simulink model "faultdetection"  (R2024b)
settings: Solver=VariableStepAuto  StartTime=0.0  StopTime=0.7  RelTol=1e-3
libraries: spsThreePhaseFaultLib x6, spsThreePhaseSourceLib x3, spsDistributedParametersLineLib x2, spsGroundLib x2, spsThreePhaseParallelRLCLoadLib x2, spsThreePhaseTransformer12TerminalsLib x2, spsThreePhaseSeriesRLCLoadLib x1, spsThreePhaseVIMeasurementLib x1, spspowerguiLib x1
settings Model: Creator=Vignesh  LastModifiedBy=Vignesh

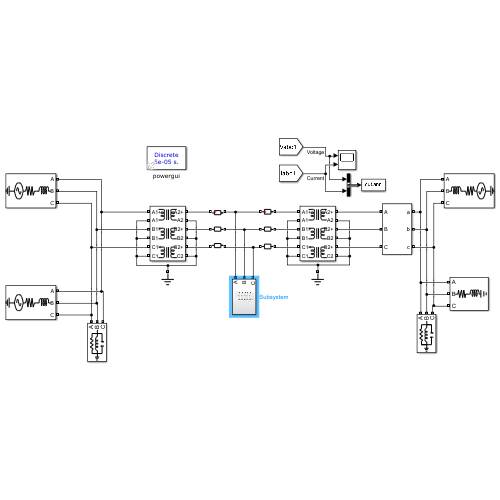
[thumbnail: Simulink's stored preview of the top-level diagram]
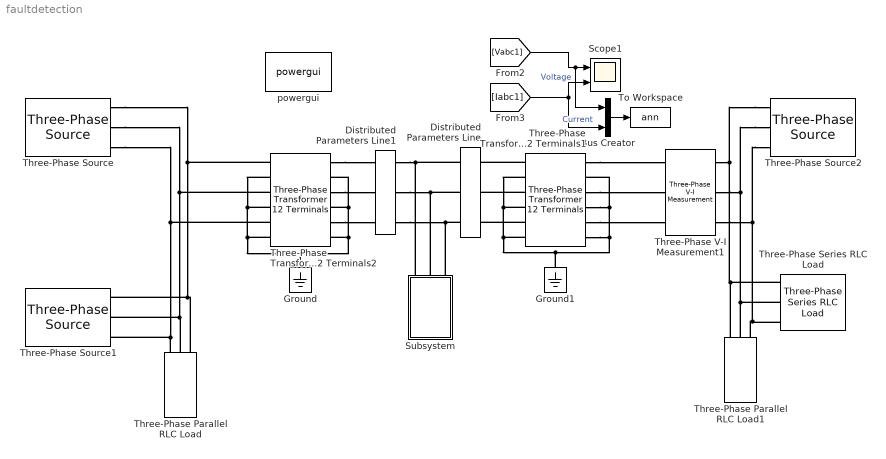
== system faultdetection ==
  Bus Creator : BusCreator  Inputs=2
  Distributed Parameters Line : spsDistributedParametersLineLib/Distributed Parameters Line  Phases=3  Length=33  Frequency=50  Resistance=[0.0132 0.132]  Inductance="[0.9337e-3  4.1264e-3]"  Capacitance=[12.74e-9 7.751e-9]  x1=[-0.0002 1.41144342231724e-10 0 0;-0.00015 1.41380923094757e-10 15635.7791244008 -78733.8101924467;-0.0001 1.41582620330545e-10 16870.5471169943 -78478.5008535494;-5e-05 1.41749384173313e-10 18101.1525545262 -78203.8281188655]  x2=[-0.0002 1.6678837341959e-10 0 0;-0.00015 1.66989876734227e-10 15586.3909292956 -78738.6897884685;-0.0001 1.67150177795504e-10 16821.2416601512 -78484.1556036395;-5e-05 1.67269237051531e-10 18051.9420013289 -78210.256627799]  x3=[-0.0002 9.38203448664615e-13 0 0;-0.00015 9.44868320985513e-13 51.7591743809092 -286.446961708197;-0.0001 9.51300061186575e-13 56.2521023005721 -285.598625681596;-5e-05 9.57497082332148e-13 60.7311508557105 -284.679822467613]  x4=[-0.0002 4.33487932405732e-13 0 0;-0.00015 4.17361641657976e-13 53.0400736803456 -296.594100248532;-0.0001 4.01132373170257e-13 57.6922279035007 -295.724392902891;-5e-05 3.84804131271731e-13 62.330147432688 -294.78171998832]  x5=0.000186628717108595  V1=[2.547e-09 1.32e+05 1.32e+05;314.2 314.2 314.2;-0.1043 0.8095 -0.7613]  V2=[2.522e-09 1.32e+05 1.32e+05;314.2 314.2 314.2;-0.1193 0.8007 -0.7701]  I1=[2.615e-12 367.2 367.2;314.2 314.2 314.2;-0.5343 0.7771 -0.7937]  I2=[5.144e-12 607 607;314.2 314.2 314.2;-0.488 0.7934 -0.7774]  nHarmo=1  Measurements=None  Decoupling=off  VsMag0=0  VrMag0=0  VsAngle0=0  VrAngle0=0  IsMag0=0  IrMag0=0  IsAngle0=0  IrAngle0=0
      settings: LibrarySourceBlock=sps_lib/Power Grid Elements/Distributed Parameters Line
  Distributed Parameters Line1 : spsDistributedParametersLineLib/Distributed Parameters Line  Phases=3  Length=33  Frequency=50  Resistance=[0.0132 0.132]  Inductance="[0.9337e-3  4.1264e-3]"  Capacitance=[12.74e-9 7.751e-9]  x1=[-0.0002 1.51351450754522e-10 0 0;-0.00015 1.51768626873871e-10 15674.3204924212 -78626.6776409923;-0.0001 1.52148356355501e-10 16907.4009652817 -78370.7761372749;-5e-05 1.52490545506846e-10 18136.3097899449 -78095.5378172326]  x2=[-0.0002 1.41144342231724e-10 0 0;-0.00015 1.41380923094757e-10 15635.7791244008 -78733.8101924467;-0.0001 1.41582620330545e-10 16870.5471169943 -78478.5008535494;-5e-05 1.41749384173313e-10 18101.1525545262 -78203.8281188655]  x3=[-0.0002 9.38648272335829e-13 0 0;-0.00015 9.45202034808867e-13 41.4228708035807 -287.645866206956;-0.0001 9.51522582823177e-13 45.9359054607534 -286.959737874603;-5e-05 9.57608356878114e-13 50.4376061206073 -286.202806520801]  x4=[-0.0002 -6.45314572399451e-13 0 0;-0.00015 -6.40074957863135e-13 63.708177517745 -294.987739785218;-0.0001 -6.34677414408614e-13 68.3337840298898 -293.950663320191;-5e-05 -6.2912327379897e-13 72.9425302033256 -292.841058927468]  x5=0.000186628717108595  V1=[2.618e-09 1.319e+05 1.319e+05;314.2 314.2 314.2;-0.1003 0.8184 -0.7524]  V2=[2.549e-09 1.32e+05 1.32e+05;314.2 314.2 314.2;-0.1043 0.8095 -0.7613]  I1=[2.387e-12 367.3 367.3;314.2 314.2 314.2;0.1434 0.7414 -0.8294]  I2=[6.175e-12 607.4 607.4;314.2 314.2 314.2;-0.4569 0.8292 -0.7416]  nHarmo=1  Measurements=None  Decoupling=off  VsMag0=0  VrMag0=0  VsAngle0=0  VrAngle0=0  IsMag0=0  IrMag0=0  IsAngle0=0  IrAngle0=0
      settings: LibrarySourceBlock=sps_lib/Power Grid Elements/Distributed Parameters Line
  Ground : spsGroundLib/Ground  LConnTagsString=a
  Ground1 : spsGroundLib/Ground  LConnTagsString=a
  Scope1 : Scope  NumInputPorts=2
  Subsystem : Subsystem
  Three-Phase Parallel RLC Load : spsThreePhaseParallelRLCLoadLib/Three-Phase Parallel RLC Load  LConnTagsString=A|B|C  Configuration=Y (grounded)  NominalVoltage=1000  Vabc=[1e3 1e3 1e3]  Vabcp=[1e3 1e3 1e3]  NominalFrequency=60  UnbalancedPower=off  ActivePower=10e4  InductivePower=100  CapacitivePower=100  Pabc=[10e3 9e3 11e3]  QLabc=[100 90 110]  QCabc=[100 90 110]  Pabcp=[10e3 9e3 11e3]  QLabcp=[100 90 110]  QCabcp=[100 90 110]  Measurements=None  LoadType=constant Z
  Three-Phase Parallel RLC Load1 : spsThreePhaseParallelRLCLoadLib/Three-Phase Parallel RLC Load  LConnTagsString=A|B|C  Configuration=Y (grounded)  NominalVoltage=1000  Vabc=[1e3 1e3 1e3]  Vabcp=[1e3 1e3 1e3]  NominalFrequency=60  UnbalancedPower=off  ActivePower=100  InductivePower=10  CapacitivePower=10  Pabc=[10e3 9e3 11e3]  QLabc=[100 90 110]  QCabc=[100 90 110]  Pabcp=[10e3 9e3 11e3]  QLabcp=[100 90 110]  QCabcp=[100 90 110]  Measurements=None  LoadType=constant Z
  Three-Phase Series RLC Load : spsThreePhaseSeriesRLCLoadLib/Three-Phase Series RLC Load  LConnTagsString=A|B|C  Configuration=Y (grounded)  NominalVoltage=11e3  Vabc=[1e3 1e3 1e3]  Vabcp=[1e3 1e3 1e3]  NominalFrequency=50  UnbalancedPower=off  ActivePower=10e6  InductivePower=100  CapacitivePower=0  Pabc=[10e3 9e3 11e3]  QLabc=[100 90 110]  QCabc=[100 90 110]  Pabcp=[10e3 9e3 11e3]  QLabcp=[100 90 110]  QCabcp=[100 90 110]  Measurements=None  LoadType=constant Z
  Three-Phase V-I Measurement1 : spsThreePhaseVIMeasurementLib/Three-Phase V-I Measurement  VoltageMeasurement=phase-to-phase  SetLabelV=on  LabelV=Vabc1  Vpu=off  VpuLL=on  CurrentMeasurement=yes  SetLabelI=on  LabelI=Iabc1  Ipu=off  Pbase=100e6  Vbase=11e3  OutputType=Complex  PhasorSimulation=off  PSBequivalent=0
  Three-Phase Source : spsThreePhaseSourceLib/Three-Phase Source  InternalConnection=Yg  VoltagePhases=off  Voltage=11e3  PhaseAngle=0  Voltage_phases=[25e3 25e3 25e3]/sqrt(3)  PhaseAngles_phases=[0 -120 +120]  Frequency=50  NonIdealSource=on  SpecifyImpedance=off  Resistance=12  Inductance=16.58e-3  ShortCircuitLevel=50e6  BaseVoltage=11e3  XRratio=7  BusType=PV  Pref=50e6  Qref=0  Prefabc=[10e3, 10e3, 10e3]  Qrefabc=[0, 0, 0]  Qmin=-inf  Qmax=inf
  Three-Phase Source1 : spsThreePhaseSourceLib/Three-Phase Source  InternalConnection=Yg  VoltagePhases=off  Voltage=11e3  PhaseAngle=0  Voltage_phases=[25e3 25e3 25e3]/sqrt(3)  PhaseAngles_phases=[0 -120 +120]  Frequency=50  NonIdealSource=on  SpecifyImpedance=off  Resistance=12  Inductance=16.58e-3  ShortCircuitLevel=50e6  BaseVoltage=11e3  XRratio=7  BusType=PV  Pref=50e6  Qref=0  Prefabc=[10e3, 10e3, 10e3]  Qrefabc=[0, 0, 0]  Qmin=-inf  Qmax=inf
  Three-Phase Source2 : spsThreePhaseSourceLib/Three-Phase Source  InternalConnection=Yg  VoltagePhases=off  Voltage=11e3  PhaseAngle=0  Voltage_phases=[25e3 25e3 25e3]/sqrt(3)  PhaseAngles_phases=[0 -120 +120]  Frequency=50  NonIdealSource=on  SpecifyImpedance=off  Resistance=8.4  Inductance=16.58e-3  ShortCircuitLevel=20e6  BaseVoltage=11e3  XRratio=7  BusType=PV  Pref=20e6  Qref=0  Prefabc=[10e3, 10e3, 10e3]  Qrefabc=[0, 0, 0]  Qmin=-inf  Qmax=inf
  Three-Phase Transformer 12 Terminals1 : spsThreePhaseTransformer12TerminalsLib/Three-Phase Transformer 12 Terminals  RatedPower=[100e6 50]  Winding1="[ 132e3 0.002  0.05 ]"  Winding2=[ 11e3 0.002 0.05]  RmXm=[ 200 200 ]
      settings: LibrarySourceBlock=|
      | sps_lib/Power Grid Elements/Three-Phase Transformer
      | 12 Terminals
  Three-Phase Transformer 12 Terminals2 : spsThreePhaseTransformer12TerminalsLib/Three-Phase Transformer 12 Terminals  RatedPower=[100e6 50]  Winding1="[ 11e3 0.002  0.05 ]"  Winding2=[ 132e3 0.002 0.05]  RmXm=[ 200 200 ]
      settings: LibrarySourceBlock=|
      | sps_lib/Power Grid Elements/Three-Phase Transformer
      | 12 Terminals
  To Workspace : ToWorkspace  VariableName=ann  SaveFormat=Structure With Time  SampleTime=-1
  powergui : spspowerguiLib/powergui  Priority=1  SimulationMode=Discrete  SampleTime=50e-6  frequency=60  Iterations=50  frequencyindice=50  Pbase=100e6  ErrMax=1e-4  UnitsV=kV  UnitsW=MW  buscounter=0  FunctionMessages=off  echomessages=off  EnableUseOfTLC=off  CurrentSourceSwitches=off  DisableSnubberDevices=off  DisableRonSwitches=off  DisableVfSwitches=off  DisplayEquations=off  AutomaticDiscreteSolvers=off  SolverType=Tustin  Interpol=off  ExternalGateDelay=off  methode=off  Ts=0  x0status=blocks  SPID=off  SwTol=0  HookPort=off  NonlinearTolerance=1e-4  nMaxIteration=100  ContinueOnMaxIteration=off  RestoreLinks=warning  ResistiveCurrentMeasurement=off  Frange=[0:2:500]  Ylog=off  Xlog=on  ShowGrid=off  save=off  variable=ZData  structure=0  ZoomFFT=off  StartTime=0.0  cycles=1  DisplayStyle=1  fundamental=60  FreqAxis=off  MaxFrequency=1000  frequencyindicesteady=1  RmsSteady=1  display=off
  wires:
  Bus Creator/1 -> To Workspace/1
  [Iabc1] -> Bus Creator/2, Scope1/2  "Current"
  [Vabc1] -> Bus Creator/1, Scope1/1  "Voltage"
  connections:
  Three-Phase Source2/RConn2 -- Three-Phase V-I Measurement1/RConn2 -- Three-Phase Series RLC Load/LConn2 -- Three-Phase Parallel RLC Load1/LConn2
  Three-Phase Transformer 12 Terminals2/LConn2 -- Ground/LConn1 -- Three-Phase Transformer 12 Terminals2/RConn6 -- Three-Phase Transformer 12 Terminals2/RConn4 -- Three-Phase Transformer 12 Terminals2/RConn2 -- Three-Phase Transformer 12 Terminals2/LConn6 -- Three-Phase Transformer 12 Terminals2/LConn4
  Three-Phase Source1/RConn1 -- Three-Phase Source/RConn1 -- Three-Phase Transformer 12 Terminals2/LConn1 -- Three-Phase Parallel RLC Load/LConn3
  Three-Phase Source2/RConn3 -- Three-Phase Series RLC Load/LConn3 -- Three-Phase Parallel RLC Load1/LConn3 -- Three-Phase V-I Measurement1/RConn3
  Distributed Parameters Line1/RConn2 -- Distributed Parameters Line/LConn2 -- Subsystem/LConn2
  Three-Phase Transformer 12 Terminals2/LConn5 -- Three-Phase Source/RConn3 -- Three-Phase Parallel RLC Load/LConn1 -- Three-Phase Source1/RConn3
  Three-Phase Transformer 12 Terminals1/RConn2 -- Ground1/LConn1 -- Three-Phase Transformer 12 Terminals1/LConn2 -- Three-Phase Transformer 12 Terminals1/LConn4 -- Three-Phase Transformer 12 Terminals1/LConn6 -- Three-Phase Transformer 12 Terminals1/RConn6 -- Three-Phase Transformer 12 Terminals1/RConn4
  Three-Phase Source2/RConn1 -- Three-Phase Series RLC Load/LConn1 -- Three-Phase Parallel RLC Load1/LConn1 -- Three-Phase V-I Measurement1/RConn1
  Subsystem/LConn3 -- Distributed Parameters Line/LConn3 -- Distributed Parameters Line1/RConn3
  Three-Phase Source1/RConn2 -- Three-Phase Source/RConn2 -- Three-Phase Transformer 12 Terminals2/LConn3 -- Three-Phase Parallel RLC Load/LConn2
  Distributed Parameters Line1/RConn1 -- Distributed Parameters Line/LConn1 -- Subsystem/LConn1
  Three-Phase Transformer 12 Terminals1/LConn3 -- Distributed Parameters Line/RConn2
  Three-Phase Transformer 12 Terminals1/LConn1 -- Distributed Parameters Line/RConn1
  Three-Phase Transformer 12 Terminals2/RConn1 -- Distributed Parameters Line1/LConn1
  Three-Phase Transformer 12 Terminals1/RConn1 -- Three-Phase V-I Measurement1/LConn1
  Three-Phase Transformer 12 Terminals1/RConn5 -- Three-Phase V-I Measurement1/LConn3
  Three-Phase Transformer 12 Terminals2/RConn3 -- Distributed Parameters Line1/LConn2
  Three-Phase Transformer 12 Terminals1/RConn3 -- Three-Phase V-I Measurement1/LConn2
  Three-Phase Transformer 12 Terminals1/LConn5 -- Distributed Parameters Line/RConn3
  Three-Phase Transformer 12 Terminals2/RConn5 -- Distributed Parameters Line1/LConn3

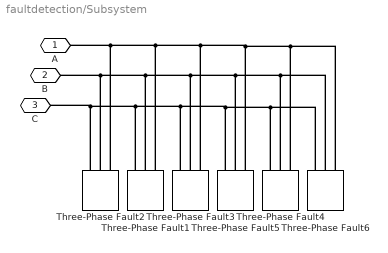
== system faultdetection/Subsystem ==
  Three-Phase Fault1 : spsThreePhaseFaultLib/Three-Phase Fault  InitialStates=0  FaultA=on  FaultB=on  FaultC=off  GroundFault=on  SwitchTimes=[ 0.3,0.35]  External=off  SwitchStatus=NaN  FaultResistance=0.001  GroundResistance=0.001  SnubberResistance=1e6  SnubberCapacitance=inf  Measurements=None
  Three-Phase Fault2 : spsThreePhaseFaultLib/Three-Phase Fault  InitialStates=0  FaultA=on  FaultB=off  FaultC=off  GroundFault=on  SwitchTimes=[ 0.1,0.15]  External=off  SwitchStatus=NaN  FaultResistance=0.001  GroundResistance=0.001  SnubberResistance=1e6  SnubberCapacitance=inf  Measurements=None
  Three-Phase Fault3 : spsThreePhaseFaultLib/Three-Phase Fault  InitialStates=0  FaultA=off  FaultB=on  FaultC=on  GroundFault=off  SwitchTimes=[ 0.2,0.25]  External=off  SwitchStatus=NaN  FaultResistance=0.001  GroundResistance=0.001  SnubberResistance=1e6  SnubberCapacitance=inf  Measurements=None
  Three-Phase Fault4 : spsThreePhaseFaultLib/Three-Phase Fault  InitialStates=0  FaultA=on  FaultB=on  FaultC=on  GroundFault=on  SwitchTimes=[ 0.5,0.55]  External=off  SwitchStatus=NaN  FaultResistance=0.001  GroundResistance=0.001  SnubberResistance=1e6  SnubberCapacitance=inf  Measurements=None
  Three-Phase Fault5 : spsThreePhaseFaultLib/Three-Phase Fault  InitialStates=0  FaultA=on  FaultB=on  FaultC=on  GroundFault=off  SwitchTimes=[ 0.4,0.45]  External=off  SwitchStatus=NaN  FaultResistance=0.001  GroundResistance=0.001  SnubberResistance=1e6  SnubberCapacitance=inf  Measurements=None
  Three-Phase Fault6 : spsThreePhaseFaultLib/Three-Phase Fault  InitialStates=0  FaultA=off  FaultB=off  FaultC=off  GroundFault=off  SwitchTimes=[ 0.02,0.05]  External=off  SwitchStatus=NaN  FaultResistance=0.001  GroundResistance=0.001  SnubberResistance=1e6  SnubberCapacitance=inf  Measurements=None
  A : PMIOPort  Side=Left
  B : PMIOPort  Port=2  Side=Left
  C : PMIOPort  Port=3  Side=Left
  connections:
  Three-Phase Fault2/LConn2 -- Three-Phase Fault6/LConn2 -- Three-Phase Fault4/LConn2 -- Three-Phase Fault5/LConn2 -- Three-Phase Fault3/LConn2 -- Three-Phase Fault1/LConn2 -- B/RConn1
  Three-Phase Fault2/LConn3 -- Three-Phase Fault6/LConn3 -- Three-Phase Fault4/LConn3 -- Three-Phase Fault5/LConn3 -- Three-Phase Fault3/LConn3 -- Three-Phase Fault1/LConn3 -- C/RConn1
  Three-Phase Fault2/LConn1 -- Three-Phase Fault6/LConn1 -- Three-Phase Fault4/LConn1 -- Three-Phase Fault5/LConn1 -- Three-Phase Fault3/LConn1 -- Three-Phase Fault1/LConn1 -- A/RConn1
